simulink model "AC_Electronic_Load"  (R2023b)
settings: Solver=FixedStepAuto  StartTime=0  StopTime=1  RelTol=1e-3
InitFcn:
  | L=680e-6;
  | C=2e-3;
  | R=0.005;
  | Cf=3e-6;
  | 
  | fc=20000;
  | Ts=1/20000;
libraries: spsSeriesRLCBranchLib x8, spsCurrentMeasurementLib x3, spsRMSLib x3, spsVoltageMeasurementLib x3, spsACVoltageSourceLib x2, spsMeanLib x2, spsUniversalBridgeLib x2, simulink x2, slpidlib x1, powerlib_extras x1, spsTHDLib x1, spspowerguiLib x1
settings Model: Creator=45276  LastModifiedBy=45276
settings DebuggingCC: SignalInfNanChecking=error  AlgebraicLoopMsg=error  BlockPriorityViolationMsg=error  UnconnectedInputMsg=warning  UnconnectedOutputMsg=warning  UnconnectedLineMsg=warning
settings ModelReferenceCC: EnableRefExpFcnMdlSchedulingChecks=on
settings RTWCC: DLArmComputeVersion=19.05

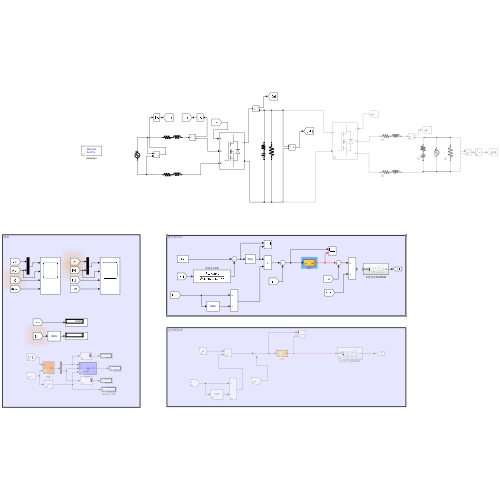
[thumbnail: Simulink's stored preview of the top-level diagram]
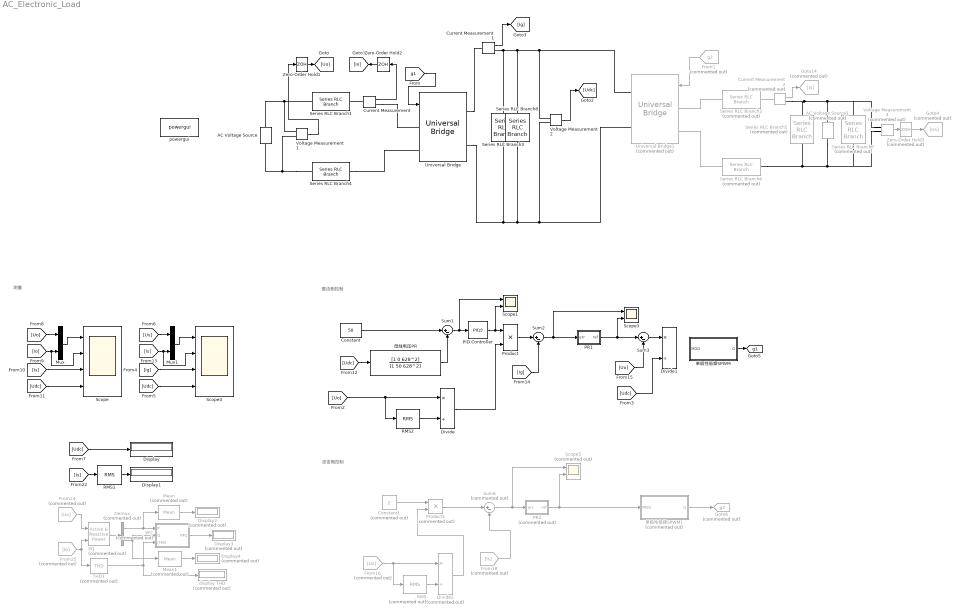
== system AC_Electronic_Load ==
  note: 逆变侧控制
  note: 整流侧控制
  note: 测量
  AC Voltage Source : spsACVoltageSourceLib/AC Voltage Source  Amplitude=30*sqrt(2)  Phase=0  Frequency=50  SampleTime=0  Measurements=None  BusType=swing  Pref=10e3  Qref=0  Qmin=-inf  Qmax=+inf
  AC Voltage Source1 : spsACVoltageSourceLib/AC Voltage Source  Commented=on  Amplitude=36*sqrt(2)  Phase=0  Frequency=50  SampleTime=0  Measurements=None  BusType=swing  Pref=10e3  Qref=0  Qmin=-inf  Qmax=+inf
  Constant : Constant  Value=50
  Constant1 : Constant  Commented=on  Value=2
  Current Measurement : spsCurrentMeasurementLib/Current Measurement  PhasorSimulation=off  OutputType=Complex  PSBequivalent=0
  Current Measurement1 : spsCurrentMeasurementLib/Current Measurement  PhasorSimulation=off  OutputType=Complex  PSBequivalent=0
  Current Measurement2 : spsCurrentMeasurementLib/Current Measurement  Commented=on  PhasorSimulation=off  OutputType=Complex  PSBequivalent=0
  Demux : Demux  Commented=on  Outputs=2
  Display : Display
  Display1 : Display
  Display2 : Display  Commented=on
  Display3 : Display  Commented=on
  Display4 : Display  Commented=on
  Divide : Product  Inputs=*/
  Divide1 : Product  Inputs=*/
  Divide2 : Product  Commented=on  Inputs=*/
  From1 : From  Commented=on  GotoTag=g2  TagVisibility=global
  From16 : From  Commented=on  GotoTag=Us
  From18 : From  Commented=on  GotoTag=Is
  From24 : From  Commented=on  GotoTag=Uo
  From25 : From  Commented=on  GotoTag=Io
  Goto14 : Goto  Commented=on  GotoTag=Is
  Goto4 : Goto  Commented=on  GotoTag=Us
  Goto6 : Goto  Commented=on  GotoTag=g2  TagVisibility=global
  Mean : spsMeanLib/Mean  Commented=on  Freq=50  Vinit=0  Ts=0
  Mean1 : spsMeanLib/Mean  Commented=on  Freq=50  Vinit=0  Ts=0
  Mux : Mux  Inputs=2
  Mux1 : Mux  Inputs=2
  PFC : MATLAB Function  Commented=on  TreatAsAtomicUnit=on
  PID Controller : slpidlib/PID Controller  Controller=PI  Form=Parallel  TimeDomain=Discrete-time  UseExternalTs=off  SampleTime=Ts  IntegratorMethod=Trapezoidal  FilterMethod=Forward Euler  ControllerParametersSource=internal  P=0.01  I=10  UseKiTs=off  D=0  N=100  UseFilter=on  TunerSelectOption=Transfer Function Based (PID Tuner App)  InitialConditionSource=internal  InitialConditionForIntegrator=0  InitialConditionForFilter=0  DifferentiatorICPrevScaledInput=0  ExternalReset=none  TrackingMode=off  Kt=1  LimitOutput=off  SatLimitsSource=internal  UpperSaturationLimit=inf  LowerSaturationLimit=-inf  LinearizeAsGain=on  AntiWindupMode=none  Kb=1  LimitIntegrator=off  UpperIntegratorSaturationLimit=inf  LowerIntegratorSaturationLimit=-inf  POutMin=[]  POutMax=[]  IOutMin=[]  IOutMax=[]  DOutMin=[]  DOutMax=[]  NOutMin=[]  NOutMax=[]  SumOutMin=[]  SumOutMax=[]  SaturationOutMin=[]  SaturationOutMax=[]  PParamMin=[]  PParamMax=[]  IParamMin=[]  IParamMax=[]  DParamMin=[]  DParamMax=[]  NParamMin=[]  NParamMax=[]  KbParamMin=[]  KbParamMax=[]  KtParamMin=[]  KtParamMax=[]  KbOutMin=[]  KbOutMax=[]  KtOutMin=[]  KtOutMax=[]  IntegratorOutMin=[]  IntegratorOutMax=[]  FilterOutMin=[]  FilterOutMax=[]  SumI1OutMin=[]  SumI1OutMax=[]  SumI2OutMin=[]  SumI2OutMax=[]  SumI3OutMin=[]  SumI3OutMax=[]  SumI4OutMin=[]  SumI4OutMax=[]  SumDOutMin=[]  SumDOutMax=[]  DifferentiatorOutMin=[]  DifferentiatorOutMax=[]  FilterDiffOutCoefMin=[]  FilterDiffOutCoefMax=[]  ReciprocalOutMin=[]  ReciprocalOutMax=[]  SumDenOutMin=[]  SumDenOutMax=[]  SumNumOutMin=[]  SumNumOutMax=[]  DivideOutMin=[]  DivideOutMax=[]  UdiffTsProdOutMin=[]  UdiffTsProdOutMax=[]  NTsProdOutMin=[]  NTsProdOutMax=[]  UintegralTsProdOutMin=[]  UintegralTsProdOutMax=[]  UngainTsProdOutMin=[]  UngainTsProdOutMax=[]  ClampingZeroOutDataTypeStr=Inherit: Inherit via back propagation  ClampingZeroOutMin=[]  ClampingZeroOutMax=[]  FilterDenConstantOutDataTypeStr=Inherit: Inherit via back propagation  FilterDenConstantOutMin=[]  FilterDenConstantOutMax=[]  PCopyOutDataTypeStr=Inherit: Inherit via back propagation  PCopyOutMin=[]  PCopyOutMax=[]  NCopyOutDataTypeStr=Inherit: Inherit via back propagation  NCopyOutMin=[]  NCopyOutMax=[]  IntegratorContinuousStateAttributes=''  IntegratorStateMustResolveToSignalObject=off  IntegratorRTWStateStorageClass=Auto  FilterContinuousStateAttributes=''  FilterStateMustResolveToSignalObject=off  FilterRTWStateStorageClass=Auto  ParallelPVariant=InternalParameters  IdealPVariant=Disabled  IVariant=InternalParameters  DVariant=Disabled  IntegratorVariant=Discrete  SatVariant=Disabled  AWVariant=Passthrough  PCopyVariant=Disabled  TRVariant=Disabled  FdbkBlocksVariant=Forward  IdealPFdbkVariant=Disabled  SatFdbkVariant=Disabled  DerivativeFilterVariant=Disabled  NVariant=Disabled  NCopyVariant=Disabled_SignalSpec  FilterICVariant=Disabled  IntegratorICVariant=InternalICs  ExternalResetVariant=Disabled  TRSumVariant=Passthrough  SumFdbkVariant=Disabled  SumVariant=Sum_PI  TsampFilterVariant=InternalTs  TsampNgainVariant=Passthrough  TsampIntegralVariant=Disabled_SignalSpec  ExternalSaturationOutDataTypeStr=Inherit: Same as second input
  PQ : powerlib_extras/Measurements/Active & Reactive Power  Commented=on  f1=50
  PR1 : Subsystem  TreatAsAtomicUnit=on  mask{Kp=4, Kr=80, Wc=5, Upper=100, Lower=-100}
  PR2 : Subsystem  Commented=on  TreatAsAtomicUnit=on  mask{Kp=4, Kr=100, Wc=5, Upper=100, Lower=-100}
  Product : Product
  Product1 : Product  Commented=on
  RMS : spsRMSLib/RMS  Commented=on  TrueRMS=off  Freq=50  RMSInit=36  Ts=0
  RMS1 : spsRMSLib/RMS  TrueRMS=off  Freq=50  RMSInit=30  Ts=0
  RMS2 : spsRMSLib/RMS  TrueRMS=off  Freq=50  RMSInit=30  Ts=0
  Scope : Scope  NumInputPorts=4
  Scope1 : Scope  NumInputPorts=2
  Scope3 : Scope  NumInputPorts=2
  Scope4 : Scope  NumInputPorts=4
  Scope5 : Scope  Commented=on  NumInputPorts=2
  Series RLC Branch1 : spsSeriesRLCBranchLib/Series RLC Branch  LConnTagsString=__new0  RConnTagsString=__new0  BranchType=RL  Resistance=R  Inductance=L  SetiL0=off  InitialCurrent=0  Capacitance=1e-6  Setx0=off  InitialVoltage=0  Measurements=None
  Series RLC Branch2 : spsSeriesRLCBranchLib/Series RLC Branch  Commented=on  LConnTagsString=__new0  RConnTagsString=__new0  BranchType=RL  Resistance=R  Inductance=L  SetiL0=off  InitialCurrent=0  Capacitance=1e-6  Setx0=off  InitialVoltage=0  Measurements=None
  Series RLC Branch3 : spsSeriesRLCBranchLib/Series RLC Branch  LConnTagsString=__new0  RConnTagsString=__new0  BranchType=RC  Resistance=0.01  Inductance=1e-3  SetiL0=off  InitialCurrent=0  Capacitance=C  Setx0=off  InitialVoltage=0  Measurements=None
  Series RLC Branch4 : spsSeriesRLCBranchLib/Series RLC Branch  LConnTagsString=__new0  RConnTagsString=__new0  BranchType=RL  Resistance=R  Inductance=L  SetiL0=off  InitialCurrent=0  Capacitance=1e-6  Setx0=off  InitialVoltage=0  Measurements=None
  Series RLC Branch5 : spsSeriesRLCBranchLib/Series RLC Branch  Commented=on  LConnTagsString=__new0  RConnTagsString=__new0  BranchType=RC  Resistance=0.002  Inductance=1e-3  SetiL0=off  InitialCurrent=0  Capacitance=Cf  Setx0=off  InitialVoltage=0  Measurements=None
  Series RLC Branch6 : spsSeriesRLCBranchLib/Series RLC Branch  Commented=on  LConnTagsString=__new0  RConnTagsString=__new0  BranchType=RL  Resistance=R  Inductance=L  SetiL0=off  InitialCurrent=0  Capacitance=1e-6  Setx0=off  InitialVoltage=0  Measurements=None
  Series RLC Branch7 : spsSeriesRLCBranchLib/Series RLC Branch  Commented=on  LConnTagsString=__new0  RConnTagsString=__new0  BranchType=R  Resistance=10  Inductance=1e-3  SetiL0=off  InitialCurrent=0  Capacitance=Cf  Setx0=off  InitialVoltage=0  Measurements=None
  Series RLC Branch8 : spsSeriesRLCBranchLib/Series RLC Branch  LConnTagsString=__new0  RConnTagsString=__new0  BranchType=R  Resistance=10  Inductance=1e-3  SetiL0=off  InitialCurrent=0  Capacitance=C  Setx0=off  InitialVoltage=0  Measurements=None
  Sum1 : Sum  Inputs=|+-
  Sum2 : Sum  Inputs=|+-
  Sum3 : Sum  Inputs=|+-
  Sum6 : Sum  Commented=on  Inputs=|+-
  THD1 : spsTHDLib/THD  Commented=on  Freq=60  Ts=0
  Universal Bridge : spsUniversalBridgeLib/Universal Bridge  Arms=2  SnubberResistance=1e5  SnubberCapacitance=inf  Device=MOSFET / Diodes  Ron=1e-2  Lon=0  ForwardVoltages="[  0  0  ]"  ForwardVoltage=0  GTOparameters=[ 10e-6 , 20e-6 ]  IGBTparameters=[ 1e-6 , 2e-6 ]  Measurements=None  Measurements_2=None  converterType=Rectifier
  Universal Bridge1 : spsUniversalBridgeLib/Universal Bridge  Commented=on  Arms=2  SnubberResistance=1e5  SnubberCapacitance=inf  Device=MOSFET / Diodes  Ron=1e-2  Lon=0  ForwardVoltages="[  0  0  ]"  ForwardVoltage=0  GTOparameters=[ 10e-6 , 20e-6 ]  IGBTparameters=[ 1e-6 , 2e-6 ]  Measurements=None  Measurements_2=None  converterType=Rectifier
  Voltage Measurement1 : spsVoltageMeasurementLib/Voltage Measurement  PhasorSimulation=off  OutputType=Complex  PSBequivalent=0
  Voltage Measurement2 : spsVoltageMeasurementLib/Voltage Measurement  PhasorSimulation=off  OutputType=Complex  PSBequivalent=0
  Voltage Measurement3 : spsVoltageMeasurementLib/Voltage Measurement  Commented=on  PhasorSimulation=off  OutputType=Complex  PSBequivalent=0
  Zero-Order Hold1 : ZeroOrderHold  SampleTime=Ts
  Zero-Order Hold2 : ZeroOrderHold  SampleTime=Ts
  Zero-Order Hold3 : ZeroOrderHold  Commented=on  SampleTime=Ts
  display THD : Display  Commented=on
  powergui : spspowerguiLib/powergui  Priority=1  SimulationMode=Discrete  SampleTime=2e-7  frequency=60  Iterations=50  frequencyindice=50  Pbase=100e6  ErrMax=1e-4  UnitsV=kV  UnitsW=MW  buscounter=0  FunctionMessages=off  echomessages=off  EnableUseOfTLC=off  CurrentSourceSwitches=off  DisableSnubberDevices=off  DisableRonSwitches=off  DisableVfSwitches=off  DisplayEquations=off  AutomaticDiscreteSolvers=off  SolverType=Tustin/Backward Euler (TBE)  Interpol=off  ExternalGateDelay=off  methode=off  Ts=100  x0status=blocks  SPID=on  SwTol=0  HookPort=off  NonlinearTolerance=1e-4  nMaxIteration=100  ContinueOnMaxIteration=off  RestoreLinks=warning  ResistiveCurrentMeasurement=off  Frange=[0:2:500]  Ylog=off  Xlog=on  ShowGrid=off  save=off  variable=ZData  structure=0  ZoomFFT=off  StartTime=0.0  cycles=1  DisplayStyle=1  fundamental=60  FreqAxis=off  MaxFrequency=1000  frequencyindicesteady=1  RmsSteady=1  display=off
  单极性倍频SPWM : Subsystem
  单极性倍频SPWM1 : Subsystem  Commented=on
  母线电压PR : TransferFcn  Numerator=[1 0 628^2]  Denominator=[1 50 628^2]
  tag scope: g1=global
  wires:
  [Udc] -> Display/1
  [Uo] -> Mux/1
  [Io] -> Scope/2, Mux/2
  Mux/1 -> Scope/1
  [Is] -> Scope/3
  [Udc] -> Scope/4
  Voltage Measurement1/1 -> Zero-Order Hold1/1
  Zero-Order Hold1/1 -> [Uo]
  Current Measurement/1 -> Zero-Order Hold2/1
  Zero-Order Hold2/1 -> [Io]
  PID Controller/1 -> Scope1/2, Product/1
  Divide/1 -> Product/2
  [Ig] -> Sum2/2
  [Uo] -> Sum3/2
  Voltage Measurement3/1 -> Zero-Order Hold3/1
  Zero-Order Hold3/1 -> Goto4/1
  Constant/1 -> Sum1/1
  Product/1 -> Sum2/1
  [Is] -> RMS1/1
  RMS1/1 -> Display1/1
  PQ/1 -> Demux/1
  Mean1/1 -> Display4/1
  From24/1 -> PQ/1
  Demux/1 -> Mean/1, PFC/1(P)
  Demux/2 -> PFC/2(Q), Mean1/1
  From25/1 -> PQ/2, THD1/1
  Mean/1 -> Display2/1
  THD1/1 -> PFC/3(iTHD), display THD/1
  Current Measurement2/1 -> Goto14/1
  PFC/1(PFC) -> Display3/1
  单极性倍频SPWM/1(G) -> [g1]
  单极性倍频SPWM1/1(G) -> Goto6/1
  [g1] -> Universal Bridge/1
  From1/1 -> Universal Bridge1/1
  [Udc] -> 母线电压PR/1
  母线电压PR/1 -> Sum1/2
  [Udc] -> Divide1/2
  Sum3/1 -> Divide1/1
  [Udc] -> Scope4/4
  [Ig] -> Scope4/3
  Mux1/1 -> Scope4/1
  [Is] -> Mux1/2, Scope4/2
  [Us] -> Mux1/1
  RMS/1 -> Divide2/2
  From16/1 -> RMS/1, Divide2/1
  Sum6/1 -> PR2/1(err), Scope5/1
  PR2/1(ref) -> 单极性倍频SPWM1/1(MOD), Scope5/2
  Constant1/1 -> Product1/1
  Divide2/1 -> Product1/2
  Product1/1 -> Sum6/1
  From18/1 -> Sum6/2
  PR1/1(ref) -> Sum3/1, Scope3/2
  Current Measurement1/1 -> [Ig]
  Voltage Measurement2/1 -> [Udc]
  Sum1/1 -> PID Controller/1, Scope1/1
  Sum2/1 -> PR1/1(err), Scope3/1
  RMS2/1 -> Divide/2
  [Uo] -> Divide/1, RMS2/1
  connections:
  AC Voltage Source/RConn1 -- Voltage Measurement1/LConn1 -- Series RLC Branch1/LConn1
  Voltage Measurement2/LConn2 -- Universal Bridge1/RConn2 -- Series RLC Branch8/RConn1 -- Series RLC Branch3/RConn1 -- Universal Bridge/RConn2
  Voltage Measurement1/LConn2 -- Series RLC Branch4/LConn1 -- AC Voltage Source/LConn1
  Current Measurement/LConn1 -- Series RLC Branch1/RConn1
  Series RLC Branch7/RConn1 -- Voltage Measurement3/LConn2 -- AC Voltage Source1/LConn1 -- Series RLC Branch6/RConn1 -- Series RLC Branch5/RConn1
  Series RLC Branch7/LConn1 -- Voltage Measurement3/LConn1 -- AC Voltage Source1/RConn1 -- Current Measurement2/RConn1 -- Series RLC Branch5/LConn1
  Series RLC Branch3/LConn1 -- Current Measurement1/RConn1 -- Series RLC Branch8/LConn1 -- Universal Bridge1/RConn1 -- Voltage Measurement2/LConn1
  Current Measurement2/LConn1 -- Series RLC Branch2/RConn1
  Current Measurement/RConn1 -- Universal Bridge/LConn1
  Series RLC Branch4/RConn1 -- Universal Bridge/LConn2
  Universal Bridge/RConn1 -- Current Measurement1/LConn1
  Universal Bridge1/LConn1 -- Series RLC Branch2/LConn1
  Universal Bridge1/LConn2 -- Series RLC Branch6/LConn1

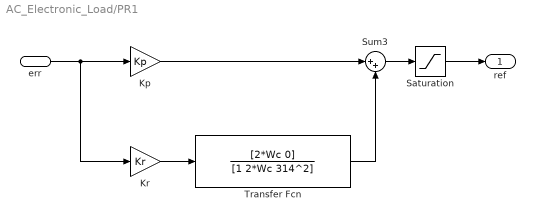
== system AC_Electronic_Load/PR1 ==
  err : Inport
  Kp : Gain  Gain=Kp
  Kr : Gain  Gain=Kr
  Saturation : Saturate  UpperLimit=Upper  LowerLimit=Lower
  Sum3 : Sum  Inputs=|++
  Transfer Fcn : TransferFcn  Numerator=[2*Wc 0]  Denominator=[1 2*Wc 314^2]
  ref : Outport
  wires:
  Saturation/1 -> ref/1
  Transfer Fcn/1 -> Sum3/2
  Kr/1 -> Transfer Fcn/1
  err/1 -> Kp/1, Kr/1
  Sum3/1 -> Saturation/1
  Kp/1 -> Sum3/1

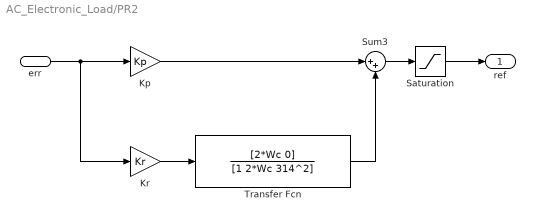
== system AC_Electronic_Load/PR2 ==
  err : Inport
  Kp : Gain  Gain=Kp
  Kr : Gain  Gain=Kr
  Saturation : Saturate  UpperLimit=Upper  LowerLimit=Lower
  Sum3 : Sum  Inputs=|++
  Transfer Fcn : TransferFcn  Numerator=[2*Wc 0]  Denominator=[1 2*Wc 314^2]
  ref : Outport
  wires:
  Kp/1 -> Sum3/1
  Sum3/1 -> Saturation/1
  err/1 -> Kr/1, Kp/1
  Kr/1 -> Transfer Fcn/1
  Transfer Fcn/1 -> Sum3/2
  Saturation/1 -> ref/1

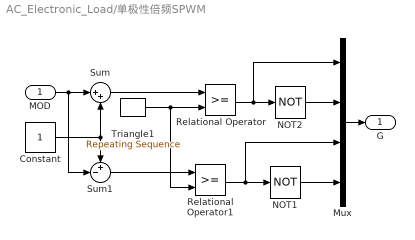
== system AC_Electronic_Load/单极性倍频SPWM ==
  MOD : Inport
  Constant : Constant
  Mux : Mux
  NOT1 : Logic  Operator=NOT  IconShape=distinctive  AllPortsSameDT=off  OutDataTypeStr=boolean
  NOT2 : Logic  Operator=NOT  IconShape=distinctive  AllPortsSameDT=off  OutDataTypeStr=boolean
  Relational Operator : RelationalOperator  OutDataTypeStr=boolean  RndMeth=Simplest  InputSameDT=off
  Relational Operator1 : RelationalOperator  OutDataTypeStr=boolean  RndMeth=Simplest  InputSameDT=off
  Sum : Sum  Inputs=|++
  Sum1 : Sum  Inputs=+-|
  Triangle1 : simulink/Sources/Repeating Sequence  rep_seq_t=[0 1/20000/2 1/20000]  rep_seq_y=[0 2 0]
  G : Outport
  wires:
  MOD/1 -> Sum1/2, Sum/1
  Mux/1 -> G/1
  Constant/1 -> Sum/2, Sum1/1
  Sum/1 -> Relational Operator/1
  Triangle1/1 -> Relational Operator1/2, Relational Operator/2
  Relational Operator/1 -> NOT2/1, Mux/1
  Sum1/1 -> Relational Operator1/1
  Relational Operator1/1 -> Mux/3, NOT1/1
  NOT1/1 -> Mux/4
  NOT2/1 -> Mux/2

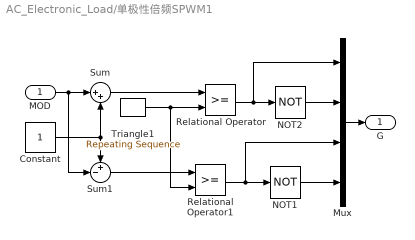
== system AC_Electronic_Load/单极性倍频SPWM1 ==
  MOD : Inport
  Constant : Constant
  Mux : Mux
  NOT1 : Logic  Operator=NOT  IconShape=distinctive  AllPortsSameDT=off  OutDataTypeStr=boolean
  NOT2 : Logic  Operator=NOT  IconShape=distinctive  AllPortsSameDT=off  OutDataTypeStr=boolean
  Relational Operator : RelationalOperator  OutDataTypeStr=boolean  RndMeth=Simplest  InputSameDT=off
  Relational Operator1 : RelationalOperator  OutDataTypeStr=boolean  RndMeth=Simplest  InputSameDT=off
  Sum : Sum  Inputs=|++
  Sum1 : Sum  Inputs=+-|
  Triangle1 : simulink/Sources/Repeating Sequence  rep_seq_t=[0 1/20000/2 1/20000]  rep_seq_y=[0 2 0]
  G : Outport
  wires:
  NOT2/1 -> Mux/2
  NOT1/1 -> Mux/4
  Relational Operator1/1 -> NOT1/1, Mux/3
  Sum1/1 -> Relational Operator1/1
  Relational Operator/1 -> Mux/1, NOT2/1
  Triangle1/1 -> Relational Operator/2, Relational Operator1/2
  Sum/1 -> Relational Operator/1
  Constant/1 -> Sum1/1, Sum/2
  Mux/1 -> G/1
  MOD/1 -> Sum/1, Sum1/2

== matlab function AC_Electronic_Load/PFC ==
  data: P input; PFC output; Q input; iTHD input
function PFC = fcn(P,Q,iTHD)
% This block supports an embeddable subset of the MATLAB language.
% See the help menu for details. 
PFC=(P/sqrt(P*P+Q*Q))/sqrt(1+iTHD^2);
